simulink model "Fuzzy_Logic"  (R2023a)
settings: Solver=VariableStepAuto  StartTime=0.0  StopTime=10  FixedStep=1E-6  RelTol=1e-3
libraries: spsDiodeLib x2, spsSeriesRLCBranchLib x2, spsMosfetLib x1, spsPVArrayLib x1, spsParallelRLCBranchLib x1, spsSeriesRLCLoadLib x1, fuzblock x1, spsPWMGeneratorDCDCLib x1, sps_lib x1
settings Model: Creator=ondetoli  LastModifiedBy=Solal
settings SolverCC: AlgebraicLoopSolver=TrustRegion
settings DebuggingCC: UnconnectedInputMsg=warning  UnconnectedOutputMsg=warning  UnconnectedLineMsg=warning
settings ModelReferenceCC: EnableRefExpFcnMdlSchedulingChecks=on
settings SFSimCC: CustomCodeUndefinedFunction=UseInterfaceOnly

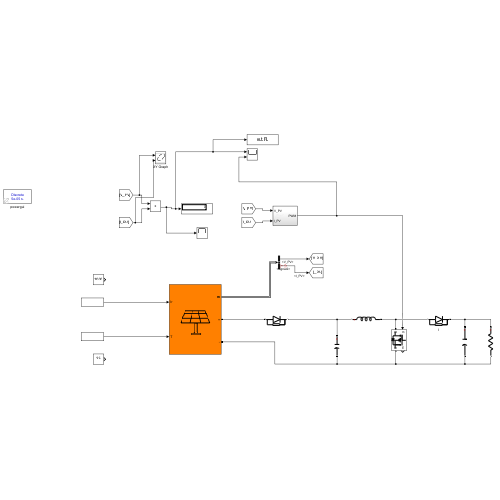
[thumbnail: Simulink's stored preview of the top-level diagram]
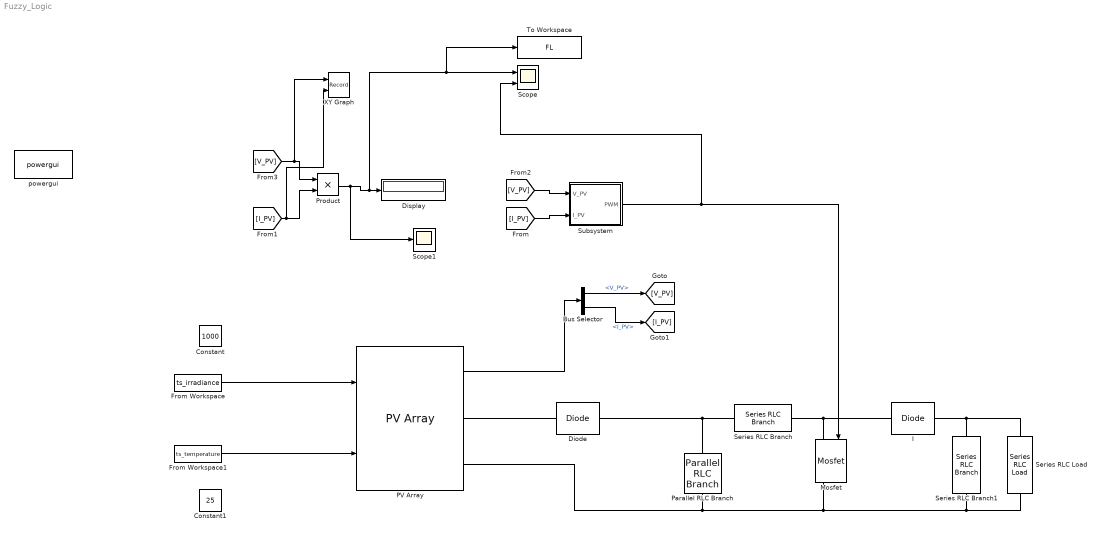
== system Fuzzy_Logic ==
  Bus Selector : BusSelector  OutputSignals=V_PV,I_PV
  Constant : Constant  Value=1000
  Constant1 : Constant  Value=25
  Diode : spsDiodeLib/Diode  Ron=0.001  Lon=0  Vf=0.8  IC=0  UseSnubber=0  Rs=500  Cs=250e-9  Measurements=off
  Display : Display
  From Workspace : FromWorkspace  VariableName=ts_irradiance
  From Workspace1 : FromWorkspace  VariableName=ts_temperature
  I : spsDiodeLib/Diode  Ron=0.001  Lon=0  Vf=0.8  IC=0  UseSnubber=0  Rs=500  Cs=250e-9  Measurements=off
  Mosfet : spsMosfetLib/Mosfet  Ron=0.1  Lon=0  Rd=0.01  Vfd=0  IC=0  Rs=1e5  Cs=inf  Measurements=on
  PV Array : spsPVArrayLib/PV Array  Npar=1  Nser=1  PlotType=one module @ 25 deg.C & specified irradiances  S_vec=1000  Temp_C_vec="[ 45 25  ]"  ModuleName=User-defined  PlotWhenSelected=off  Pm=200.143  Ncell=54  Voc=32.9  Isc=8.21  Vm=26.3  Im=7.61  beta_Voc_pc=-0.37  alpha_Isc_pc=0.0389  beta_Voc=-0.12173  alpha_Isc=0.0031937  IL=8.2275  I0=3.7751e-10  nI=0.99725  Rsh=158.0683  Rs=0.3374  RobustModel=off  RobustCellTemperature=313.3991  BAL=on  Tc=1e-6  Tfilter=5e-5
  Parallel RLC Branch : spsParallelRLCBranchLib/Parallel RLC Branch  LConnTagsString=a  RConnTagsString=__new0  BranchType=C  Resistance=1  Inductance=1e-3  SetiL0=off  InitialCurrent=0  Capacitance=4000e-6  Setx0=off  InitialVoltage=0  Measurements=None
  Product : Product
  Scope : Scope  NumInputPorts=2
  Scope1 : Scope
  Series RLC Branch : spsSeriesRLCBranchLib/Series RLC Branch  LConnTagsString=__new0  RConnTagsString=__new0  BranchType=L  Resistance=1  Inductance=4e-4  SetiL0=off  InitialCurrent=0  Capacitance=1e-6  Setx0=off  InitialVoltage=0  Measurements=None
  Series RLC Branch1 : spsSeriesRLCBranchLib/Series RLC Branch  LConnTagsString=__new0  RConnTagsString=__new0  BranchType=C  Resistance=1  Inductance=1e-3  SetiL0=off  InitialCurrent=0  Capacitance=50e-6  Setx0=off  InitialVoltage=0  Measurements=None
  Series RLC Load : spsSeriesRLCLoadLib/Series RLC Load  LConnTagsString=a  RConnTagsString=__new0  NominalVoltage=32.9  NominalFrequency=50  ActivePower=200  InductivePower=0  CapacitivePower=0  Setx0=off  InitialVoltage=0  SetiL0=off  InitialCurrent=0  Measurements=None  LoadType=constant Z
  Subsystem : Subsystem
  To Workspace : ToWorkspace  VariableName=FL  SaveFormat=Timeseries  SampleTime=-1
  XY Graph : Record  FileSettingsInternal="{\"entries\":[{\"content\":{\"excelSettings\":{\"content\":{},\"type\":\"Streamout.ExcelSettings\"}},\"type\":\"Streamout.FileSettingStorage\",\"uuid\":\"\"}],\"packageUris\":[\"http:\\/\\/schema.mathworks.com\\/mf0\\/streamout_blocks\\/R2020a\"],\"version\":\"1.0\"}"  Layout=[1 1]  SignalsInternal="{\"entries\":[{\"content\":{\"signals\":[{\"content\":{\"blockPath\":[],\"dimensions\":[1],\"domain\":\"\",\"lineColor\":\"#a2142f\",\"plots\":[1],\"port\":1,\"sid\":[\"\"],\"signalID\":4363,\"signalName\":\"From3\"},\"type\":\"RecordBlkView.Signal\",\"uuid\":\"\"},{\"content\":{\"blockPath\":[],\"dimensions\":[1],\"domain\":\"\",\"lineColor\":\"#139fff\",\"plots\":[1],\"port\":2,\"sid\":[\"\"],\"signalID\":4367,\"signalName\":\"From1\"},\"type\":\"RecordBlkView.Signal\",\"uuid\":\"\"}]},\"type\":\"RecordBlkView.InputSignals\",\"uuid\":\"\"}],\"packageUris\":[\"http:\\/\\/schema.mathworks.com\\/mf0\\/streamout_blocks\\/R2020a\"],\"version\":\"1.0\"}"  VisualizationBindings="{\"xyplotplugin\":{\"info\":[{\"series\":[{\"bindingParametersList\":[{\"parameter\":\"X-Axis\",\"signalID\":4363,\"signalName\":\"From3\"},{\"parameter\":\"Y-Axis\",\"signalID\":4367,\"signalName\":\"From1\"}],\"seriesID\":21330}],\"subplotID\":1}]}}"  CompatibilityTag=XY  st=-1
  powergui : sps_lib/powergui  Priority=1  SimulationMode=Discrete  SampleTime=50e-6  frequency=60  Iterations=50  frequencyindice=0  Pbase=100e6  ErrMax=1e-4  UnitsV=kV  UnitsW=MW  buscounter=0  FunctionMessages=off  echomessages=off  EnableUseOfTLC=off  CurrentSourceSwitches=off  DisableSnubberDevices=off  DisableRonSwitches=off  DisableVfSwitches=off  DisplayEquations=off  AutomaticDiscreteSolvers=off  SolverType=Tustin/Backward Euler (TBE)  Interpol=off  ExternalGateDelay=off  methode=off  Ts=100  x0status=blocks  SPID=on  SwTol=0  HookPort=off  NonlinearTolerance=1e-4  nMaxIteration=100  ContinueOnMaxIteration=off  RestoreLinks=warning  ResistiveCurrentMeasurement=off  Frange=[0:2:500]  Ylog=off  Xlog=on  ShowGrid=off  save=off  variable=ZData  structure=0  ZoomFFT=off  StartTime=0.0  cycles=1  DisplayStyle=1  fundamental=60  FreqAxis=off  MaxFrequency=1000  frequencyindicesteady=1  RmsSteady=1  display=off
  wires:
  PV Array/1 -> Bus Selector/1
  ? -> ?  "<signal2>"
  Bus Selector/1 -> [V_PV]  "<V_PV>"
  Bus Selector/2 -> [I_PV]  "<I_PV>"
  [V_PV] -> Subsystem/1(V_PV)
  [I_PV] -> Subsystem/2(I_PV)
  Subsystem/1(PWM) -> Scope/2, Mosfet/1
  [V_PV] -> XY Graph/1, Product/1
  [I_PV] -> XY Graph/2, Product/2
  Product/1 -> Scope1/1, To Workspace/1, Scope/1, Display/1
  From Workspace1/1 -> PV Array/2
  From Workspace/1 -> PV Array/1
  connections:
  Diode/LConn1 -- PV Array/RConn1
  PV Array/RConn2 -- Series RLC Load/RConn1 -- Series RLC Branch1/RConn1 -- Mosfet/RConn1 -- Parallel RLC Branch/RConn1
  Parallel RLC Branch/LConn1 -- Series RLC Branch/LConn1 -- Diode/RConn1
  Series RLC Branch/RConn1 -- Mosfet/LConn1 -- I/LConn1
  I/RConn1 -- Series RLC Load/LConn1 -- Series RLC Branch1/LConn1

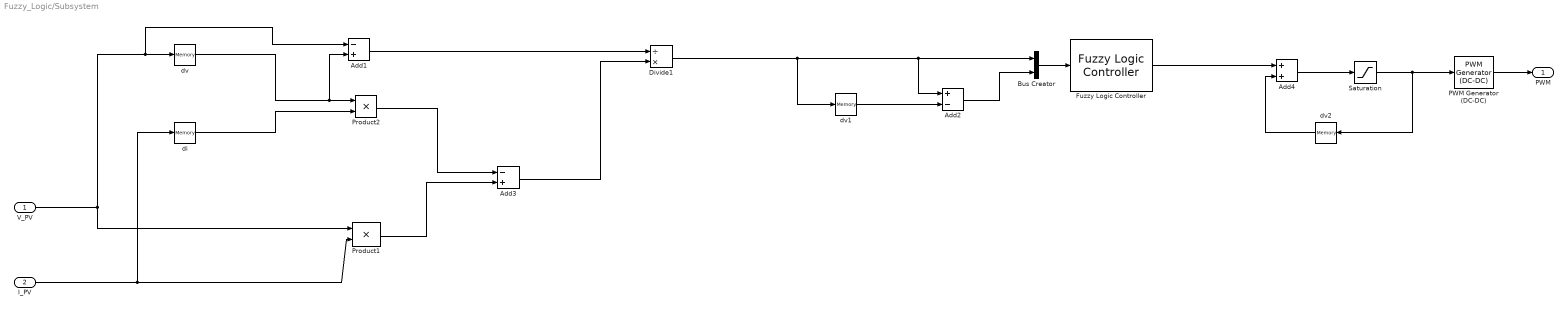
== system Fuzzy_Logic/Subsystem ==
  V_PV : Inport
  I_PV : Inport  Port=2
  Add1 : Sum  Inputs=-+
  Add2 : Sum  Inputs=+-
  Add3 : Sum  Inputs=-+
  Add4 : Sum
  Bus Creator : BusCreator  Inputs=2
  Divide1 : Product  Inputs=/*
  Fuzzy Logic Controller : fuzblock/Fuzzy Logic  Controller  FIS=x  OutputSampleNumber=101  DataType=double  FuzzifiedInputs=off  RuleFiringStrengths=off  RuleOutputs=off  AggregatedOutputs=off  SimulateUsing=Interpreted execution  OutOfRangeInputValueMessage=warning  NoRuleFiredMessage=warning  EmptyOutputFuzzySetMessage=warning
  PWM Generator (DC-DC) : spsPWMGeneratorDCDCLib/PWM Generator (DC-DC)  Fsw=15000  Ts=0
  Product1 : Product  Inputs=**
  Product2 : Product  Inputs=**
  Saturation : Saturate  UpperLimit=0.95  LowerLimit=0.1
  di : Memory
  dv : Memory
  dv1 : Memory
  dv2 : Memory
  PWM : Outport
  wires:
  Divide1/1 -> dv1/1, Bus Creator/1, Add2/1
  V_PV/1 -> Add1/1, dv/1, Product1/1
  I_PV/1 -> di/1, Product1/2
  Product1/1 -> Add3/2
  Product2/1 -> Add3/1
  di/1 -> Product2/2
  dv/1 -> Add1/2, Product2/1
  Add1/1 -> Divide1/1
  Add3/1 -> Divide1/2
  dv1/1 -> Add2/2
  Add2/1 -> Bus Creator/2
  Bus Creator/1 -> Fuzzy Logic Controller/1
  Fuzzy Logic Controller/1 -> Add4/1
  Add4/1 -> Saturation/1
  Saturation/1 -> PWM Generator (DC-DC)/1, dv2/1
  dv2/1 -> Add4/2
  PWM Generator (DC-DC)/1 -> PWM/1
